simulink subsystem "Vehicle1D_refsub_Basic"  (R2023a)
settings: Solver=VariableStepAuto  StartTime=0.0  StopTime=10.0  RelTol=1e-3
undefined symbols (not defined in the file or in its folder): vehicle
libraries: nesl_utility x6, sdl_lib x1, fl_lib x1
settings Model: Creator=isaacito  LastModifiedBy=isaacito
settings SolverCC: AlgebraicLoopSolver=TrustRegion
settings OptimizationCC: ReuseModelBlockBuffer=off
settings DebuggingCC: UnconnectedInputMsg=warning  UnconnectedOutputMsg=warning  UnconnectedLineMsg=warning
settings ModelReferenceCC: EnableRefExpFcnMdlSchedulingChecks=on
settings RTWCC: DLArmComputeVersion=19.05

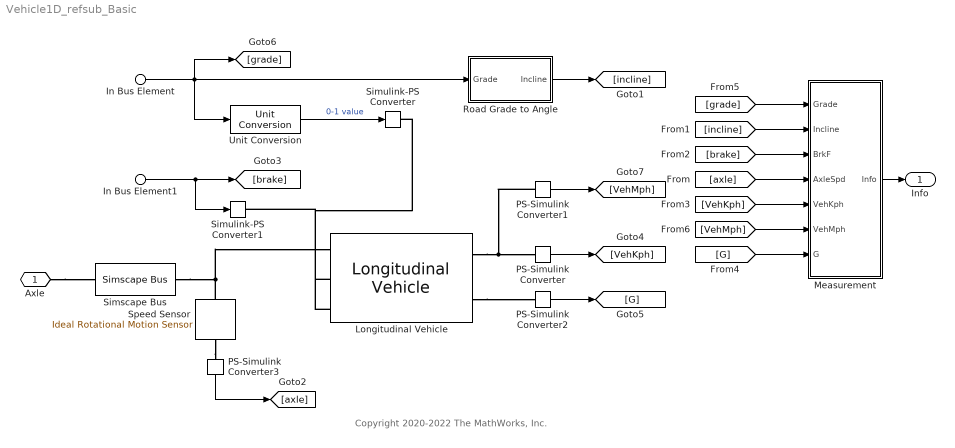
== system Vehicle1D_refsub_Basic ==
  note: Copyright 2020-2022 The MathWorks, Inc.
  In Bus Element : Inport  PortName=Inputs  Element=RoadGrade
      settings: AttributesFormatString=%<Unit>
  In Bus Element1 : Inport  PortName=Inputs  Element=BrakeForce
      settings: AttributesFormatString=%<Unit>
  Longitudinal Vehicle : sdl_lib/Tires & Vehicles/Longitudinal Vehicle  vehParamType=sdl.enum.VehicleParameterizationType.RoadLoad  M_vehicle=vehicle.mass_kg kg  R_tireroll=vehicle.tireRollingRadius_m m  C_tireroll=0.0136  C_airdrag=0.31  A_front=2.3 m^2  A_rl=vehicle.roadLoadA_N N  B_rl=vehicle.roadLoadB_N_per_kph N/(km/hr)  C_rl=vehicle.roadLoadC_N_per_kph2 N/(km/hr)^2  g=vehicle.roadLoad_gravAccel_m_per_s2 m/s^2  V_1=smoothing.vehicle_speedThreshold_kph km/hr  w_1=smoothing.vehicle_axleSpeedThreshold_rpm rpm  ShowBrakeIn=simscape.enum.onoff.on  ShowSlopeIn=simscape.enum.onoff.on  SlopeInputType=sdl.enum.VehicleLongitudinalRoadSlopeInputType.Grade  ShowWindIn=simscape.enum.onoff.off  ShowGOut=simscape.enum.onoff.on  air_density=1.184 kg/m^3  V_x_specify=on  V_x_priority=High  V_x=initial.vehicle_speed_kph km/hr  V_x_nominal_specify=off  V_x_nominal_unit=m/s  V_x_nominal_value=1  trq_specify=off  trq_priority=None  trq=0 N*m  trq_nominal_specify=off  trq_nominal_unit=N*m  trq_nominal_value=1  w_specify=off  w_priority=None  w=0 rad/s  w_nominal_specify=off  w_nominal_unit=rad/s  w_nominal_value=1
      settings: InternalSimscapePortConfiguration="{\"Bottom\":[],\"Left\":[{\"id\":\"Axle\",\"label\":\"Axle\",\"type\":\"foundation.mechanical.rotational.rotational\"}],\"Right\":[{\"id\":\"v_out\",\"label\":\"VehSpd\",\"type\":\"output\"},{\"id\":\"G_out\",\"label\":\"G\",\"type\":\"output\"}],\"Top\":[{\"id\":\"brkF\",\"label\":\"Brake\",\"type\":\"input\"},{\"id\":\"grade_norm\",\"label\":\"NG\",\"type\":\"input\"}]}"
      settings: AttributesFormatString=|
      | %<V_x> [%<V_x_unit>]
      | Priority: %<V_x_priority>
  Measurement : Subsystem
  PS-Simulink Converter : nesl_utility/PS-Simulink Converter  PhysicalDomain=network_engine_domain  SubClassName=ps_output  LeftPortType=input  RightPortType=output  PseudoPeriodic=off  Frequencies=[]  VectorFormat=1-D array  Unit=km/hr  AffineConversion=off
  PS-Simulink Converter1 : nesl_utility/PS-Simulink Converter  PhysicalDomain=network_engine_domain  SubClassName=ps_output  LeftPortType=input  RightPortType=output  PseudoPeriodic=off  Frequencies=[]  VectorFormat=1-D array  Unit=mph  AffineConversion=off
  PS-Simulink Converter2 : nesl_utility/PS-Simulink Converter  PhysicalDomain=network_engine_domain  SubClassName=ps_output  LeftPortType=input  RightPortType=output  PseudoPeriodic=off  Frequencies=[]  VectorFormat=1-D array  Unit=1  AffineConversion=off
  PS-Simulink Converter3 : nesl_utility/PS-Simulink Converter  PhysicalDomain=network_engine_domain  SubClassName=ps_output  LeftPortType=input  RightPortType=output  PseudoPeriodic=off  Frequencies=[]  VectorFormat=1-D array  Unit=rpm  AffineConversion=off
  Road Grade to Angle : Subsystem
  Simscape Bus : SimscapeBus  HierarchyStrings=AngSpd  ConnectionType=Bus: Bus_Rotational
      settings: AttributesFormatString=%<ConnectionType>
  Simulink-PS Converter : nesl_utility/Simulink-PS Converter  PhysicalDomain=network_engine_domain  SubClassName=ps_input  LeftPortType=input  RightPortType=output  PseudoPeriodic=off  Frequencies=[]  NoiseDistribution=none  NoiseParameters=[]  Unit=1  AffineConversion=off  FilteringAndDerivatives=filter  SimscapeFilterOrder=1  InputFilterTimeConstant=0.001  UdotUserProvided=0
  Simulink-PS Converter1 : nesl_utility/Simulink-PS Converter  PhysicalDomain=network_engine_domain  SubClassName=ps_input  LeftPortType=input  RightPortType=output  PseudoPeriodic=off  Frequencies=[]  NoiseDistribution=none  NoiseParameters=[]  Unit=N  AffineConversion=off  FilteringAndDerivatives=filter  SimscapeFilterOrder=1  InputFilterTimeConstant=0.001  UdotUserProvided=0
  Speed Sensor : fl_lib/Mechanical/Mechanical Sensors/Ideal Rotational Motion Sensor  reference=foundation.enum.MeasurementReference.absolute  acceleration_port=false  velocity_port=true  position_port=false  wrap_angle=simscape.enum.onoff.off  offset=0 rad
      settings: InternalSimscapePortConfiguration="{\"Bottom\":[],\"Left\":[{\"id\":\"R\",\"label\":\"R\",\"type\":\"foundation.mechanical.rotational.rotational\"}],\"Right\":[{\"id\":\"W\",\"label\":\"W\",\"type\":\"output\"}],\"Top\":[]}"
  Unit Conversion : UnitConversion  OutputType=Inherit: Inherit via back propagation
  Axle : PMIOPort  Side=Left
  Info : Outport
  wires:
  PS-Simulink Converter3/1 -> [axle]
  [incline] -> Measurement/2(Incline)
  [brake] -> Measurement/3(BrkF)
  [grade] -> Measurement/1(Grade)
  [G] -> Measurement/7(G)
  [VehKph] -> Measurement/5(VehKph)
  [axle] -> Measurement/4(AxleSpd)
  Road Grade to Angle/1(Incline) -> [incline]
  Unit Conversion/1 -> Simulink-PS Converter/1  "0-1 value"
  In Bus Element1/1 -> [brake], Simulink-PS Converter1/1
  In Bus Element/1 -> Road Grade to Angle/1(Grade), Unit Conversion/1, [grade]
  PS-Simulink Converter2/1 -> [G]
  PS-Simulink Converter/1 -> [VehKph]
  PS-Simulink Converter1/1 -> [VehMph]
  [VehMph] -> Measurement/6(VehMph)
  Measurement/1(Info) -> Info/1
  connections:
  PS-Simulink Converter1/LConn1 -- Longitudinal Vehicle/RConn1 -- PS-Simulink Converter/LConn1
  Speed Sensor/LConn1 -- Simscape Bus/LConn1 -- Longitudinal Vehicle/LConn1
  Speed Sensor/RConn1 -- PS-Simulink Converter3/LConn1
  Longitudinal Vehicle/LConn2 -- Simulink-PS Converter1/RConn1
  Longitudinal Vehicle/LConn3 -- Simulink-PS Converter/RConn1
  Longitudinal Vehicle/RConn2 -- PS-Simulink Converter2/LConn1
  Axle/RConn1 -- Simscape Bus/RConn1

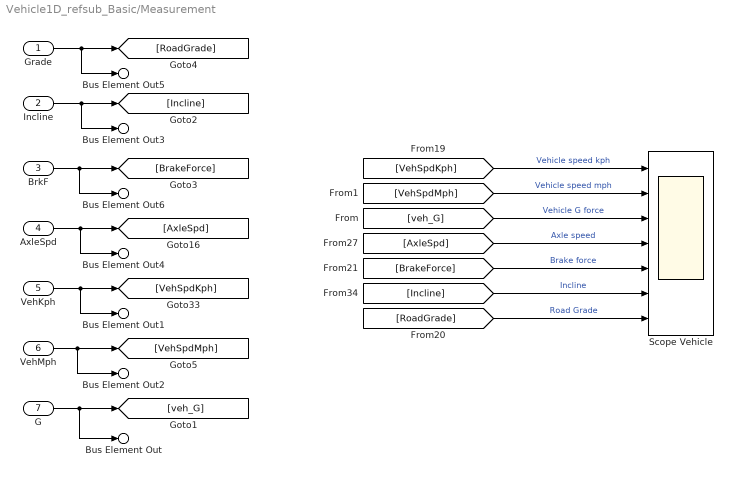
== system Vehicle1D_refsub_Basic/Measurement ==
  Grade : Inport  Unit=%
      settings: AttributesFormatString=%<Unit>
  Incline : Inport  Port=2  Unit=deg
      settings: AttributesFormatString=%<Unit>
  BrkF : Inport  Port=3  Unit=N
      settings: AttributesFormatString=%<Unit>
  AxleSpd : Inport  Port=4  Unit=rpm
      settings: AttributesFormatString=%<Unit>
  VehKph : Inport  Port=5  Unit=km/hr
      settings: AttributesFormatString=%<Unit>
  VehMph : Inport  Port=6  Unit=mph
      settings: AttributesFormatString=%<Unit>
  G : Inport  Port=7  Unit=1
      settings: AttributesFormatString=%<Unit>
  Scope Vehicle : Scope  NumInputPorts=7
  Bus Element Out : Outport  PortName=Info  Element=G
      settings: AttributesFormatString=%<Unit>
  Bus Element Out1 : Outport  PortName=Info  Element=VehSpdKph
      settings: AttributesFormatString=%<Unit>
  Bus Element Out2 : Outport  PortName=Info  Element=VehSpdMph
      settings: AttributesFormatString=%<Unit>
  Bus Element Out3 : Outport  PortName=Info  Element=Incline
      settings: AttributesFormatString=%<Unit>
  Bus Element Out4 : Outport  PortName=Info  Element=AxleSpd
      settings: AttributesFormatString=%<Unit>
  Bus Element Out5 : Outport  PortName=Info  Element=Grade
      settings: AttributesFormatString=%<Unit>
  Bus Element Out6 : Outport  PortName=Info  Element=BrkF
      settings: AttributesFormatString=%<Unit>
  wires:
  [VehSpdMph] -> Scope Vehicle/2  "Vehicle speed mph"
  VehMph/1 -> [VehSpdMph], Bus Element Out2/1
  Grade/1 -> [RoadGrade], Bus Element Out5/1
  [RoadGrade] -> Scope Vehicle/7  "Road Grade"
  [Incline] -> Scope Vehicle/6  "Incline"
  [BrakeForce] -> Scope Vehicle/5  "Brake force"
  [AxleSpd] -> Scope Vehicle/4  "Axle speed"
  BrkF/1 -> [BrakeForce], Bus Element Out6/1
  Incline/1 -> [Incline], Bus Element Out3/1
  G/1 -> [veh_G], Bus Element Out/1
  VehKph/1 -> [VehSpdKph], Bus Element Out1/1
  AxleSpd/1 -> [AxleSpd], Bus Element Out4/1
  [veh_G] -> Scope Vehicle/3  "Vehicle G force"
  [VehSpdKph] -> Scope Vehicle/1  "Vehicle speed kph"

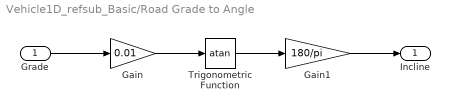
== system Vehicle1D_refsub_Basic/Road Grade to Angle ==
  Grade : Inport  Unit=%
      settings: AttributesFormatString=%<Unit>
  Gain : Gain  Gain=0.01
  Gain1 : Gain  Gain=180/pi
  Trigonometric Function : Trigonometry  Operator=atan
  Incline : Outport  Unit=deg
      settings: AttributesFormatString=%<Unit>
  wires:
  Gain/1 -> Trigonometric Function/1
  Grade/1 -> Gain/1
  Trigonometric Function/1 -> Gain1/1
  Gain1/1 -> Incline/1
